simulink model "ex_model_comparison"  (R2026b)
settings: Solver=ode23t  StopTime=2  MaxStep=1e-4  RelTol=1e-5
undefined symbols (not defined in the file or in its folder): L1, L2, L3, Rechtsdrehfeld
libraries: asm_blocks_lib x26, nesl_utility x2
settings Model: Creator=fsbb  LastModifiedBy=fsbb
settings SimscapeCC: SimscapeLogType=all  SimscapeNominalValues="[{\"value\":\"1\",\"unit\":\"A\"},{\"value\":\"1\",\"unit\":\"bar\"},{\"value\":\"1\",\"unit\":\"cm^2\"},{\"value\":\"1\",\"unit\":\"cm^3/s\"},{\"value\":\"1\",\"unit\":\"kJ/kg\"},{\"value\":\"1\",\"unit\":\"kW\"},{\"value\":\"1\",\"unit\":\"l\"},{\"value\":\"1\",\"unit\":\"N\"},{\"value\":\"1\",\"unit\":\"N*m\"},{\"value\":\"1\",\"unit\":\"V\"},{\"value\":\"0.001\",\"unit\":\"Wb\"}]"  SimscapeUseEnergyAccounting=off

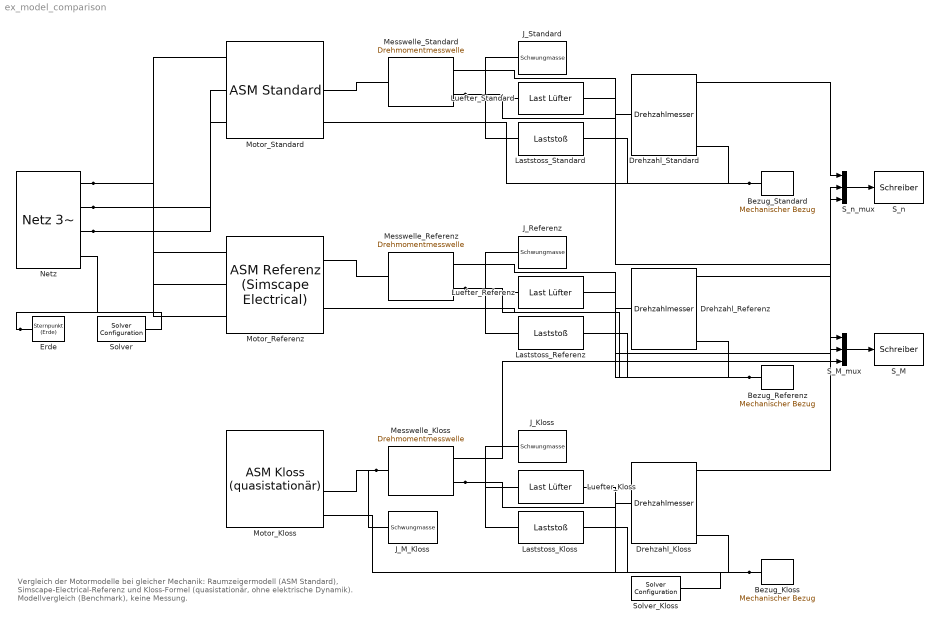
== system ex_model_comparison ==
  note: Vergleich der Motormodelle bei gleicher Mechanik: Raumzeigermodell (ASM Standard), Simscape-Electrical-Referenz und Kloss-Formel (quasistationär, ohne elektrische Dynamik). Modellvergleich (Benchmark), keine Messung.
  Bezug_Kloss : asm_blocks_lib/Mechanik/Mechanischer Bezug  Tag=asmlib:mech_reference
  Bezug_Referenz : asm_blocks_lib/Mechanik/Mechanischer Bezug  Tag=asmlib:mech_reference
  Bezug_Standard : asm_blocks_lib/Mechanik/Mechanischer Bezug  Tag=asmlib:mech_reference
  Drehzahl_Kloss : asm_blocks_lib/Messgeräte/Drehzahlmesser  Tag=asmlib:speed_sensor  ns=1500
  Drehzahl_Referenz : asm_blocks_lib/Messgeräte/Drehzahlmesser  Tag=asmlib:speed_sensor  ns=1500
  Drehzahl_Standard : asm_blocks_lib/Messgeräte/Drehzahlmesser  Tag=asmlib:speed_sensor  ns=1500
  Erde : asm_blocks_lib/Quellen/Sternpunkt (Erde)  Tag=asmlib:neutral_ground
  J_Kloss : asm_blocks_lib/Mechanik/Schwungmasse  Tag=asmlib:inertia  J=0.01  n0=0
  J_M_Kloss : asm_blocks_lib/Mechanik/Schwungmasse  Tag=asmlib:inertia  J=0.012  n0=0
  J_Referenz : asm_blocks_lib/Mechanik/Schwungmasse  Tag=asmlib:inertia  J=0.01  n0=0
  J_Standard : asm_blocks_lib/Mechanik/Schwungmasse  Tag=asmlib:inertia  J=0.01  n0=0
  Laststoss_Kloss : asm_blocks_lib/Mechanik/Laststoß  Tag=asmlib:load_step  t_step=1  dM_L=7.95
  Laststoss_Referenz : asm_blocks_lib/Mechanik/Laststoß  Tag=asmlib:load_step  t_step=1  dM_L=7.95
  Laststoss_Standard : asm_blocks_lib/Mechanik/Laststoß  Tag=asmlib:load_step  t_step=1  dM_L=7.95
  Luefter_Kloss : asm_blocks_lib/Mechanik/Last Lüfter  Tag=asmlib:load_fan  M_B=26.5  n_B=1440
  Luefter_Referenz : asm_blocks_lib/Mechanik/Last Lüfter  Tag=asmlib:load_fan  M_B=26.5  n_B=1440
  Luefter_Standard : asm_blocks_lib/Mechanik/Last Lüfter  Tag=asmlib:load_fan  M_B=26.5  n_B=1440
  Messwelle_Kloss : asm_blocks_lib/Messgeräte/Drehmomentmesswelle  Tag=asmlib:torque_sensor
  Messwelle_Referenz : asm_blocks_lib/Messgeräte/Drehmomentmesswelle  Tag=asmlib:torque_sensor
  Messwelle_Standard : asm_blocks_lib/Messgeräte/Drehmomentmesswelle  Tag=asmlib:torque_sensor
  Motor_Kloss : asm_blocks_lib/Referenz/ASM Kloss (quasistationär)  Tag=asmlib:asm_kloss  MK=71.55  sK=0.2  ns=1500
  Motor_Referenz : asm_blocks_lib/Referenz/ASM Referenz (Simscape Electrical)  Tag=asmlib:asm_reference  param_set=Standard  U_N=400  f_N=50  p=2  R1=0.5  L1s=0.009902  Lh=0.25  R2b=1.225  L2sb=0.009902  J_M=0.012
  Motor_Standard : asm_blocks_lib/Maschine/ASM Standard  Tag=asmlib:asm_standard  param_set=Standard  connection=Stern  U_N=400  f_N=50  p=2  R1=0.5  L1s=0.009902  Lh=0.25  R2b=1.225  L2sb=0.009902  J_M=0.012  k_R=0  n0=0  l=0.15  r=0.06  N2=28  Bhat_N=0.8
  Netz : asm_blocks_lib/Quellen/Netz 3~  Tag=asmlib:grid3  U_L=400  f1=50  phase_seq=L1-L2-L3 (Rechtsdrehfeld)  phi0=0  t_on=0  R_N=0  L_N=0
  S_M : asm_blocks_lib/Messgeräte/Schreiber  Tag=asmlib:recorder  title_text=Wellenmoment: Standard / Referenz / Kloss
  S_M_mux : Mux  Inputs=3
  S_n : asm_blocks_lib/Messgeräte/Schreiber  Tag=asmlib:recorder  title_text=Drehzahl: Standard / Referenz / Kloss
  S_n_mux : Mux  Inputs=3
  Solver : nesl_utility/Solver Configuration  PhysicalDomain=network_engine_domain  SubClassName=solver  LeftPortType=input  RightPortType=generic  Tones=[]  Harmonics=[]  SimulateNoise=off  Profile=off  UseLocalSampling=off  EnableSwitchedLinearOptims=on  FrequencyDomain=off  UseCCode=off  RelTol=0.001  AbsTol=0.001  MinStep=1e-09  ToWorkspace=off  RevertToSquareIcSolve=off  NumHomotopyIterations=100  PhasorMode=off  PhasorModeNumHarmonics=1  ConsistencySolver=NEWTON_XTOL_AFTER_FTOL  CanonicalOrdering=CANONICAL  OptimizeIntermediates=OPTIMIZED  MulticoreSolverChoice=BACKWARD_EULER  IndexReductionMethod=DerivativeReplacement  DoDC=off  ResidualTolerance=1e-09  ConsistencyTolSource=GLOBAL  ConsistencyAbsTol=0.001  ConsistencyRelTol=0.001  ConsistencyTolFactor=0.001  UseLocalSolver=off  LocalSolverChoice=NE_BACKWARD_EULER_ADVANCER  ResolveIndetEquations=on  FunctionEvalNumThread=1  LocalSolverSampleTime=0.001  DoFixedCost=off  MaxNonlinIter=3  MaxModeIter=2  ComputeImpulses=off  ImpulseIterations=2  LinearAlgebra=auto  LinearAlgebraNumThread=0  EquationFormulation=NE_TIME_EF  DelaysMemoryBudget=1024  AutomaticFiltering=on  FilteringTimeConstant=0.001  PartitionStorageMethod=AS_NEEDED  PartitionMemoryBudget=1024  PartitionMethod=BALANCED  MultibodyUseLocalSolver=off  MultibodyLocalSolverChoice=ODE1  MultibodyLocalSolverSampleTime=0.001
  Solver_Kloss : nesl_utility/Solver Configuration  PhysicalDomain=network_engine_domain  SubClassName=solver  LeftPortType=input  RightPortType=generic  Tones=[]  Harmonics=[]  SimulateNoise=off  Profile=off  UseLocalSampling=off  EnableSwitchedLinearOptims=on  FrequencyDomain=off  UseCCode=off  RelTol=0.001  AbsTol=0.001  MinStep=1e-09  ToWorkspace=off  RevertToSquareIcSolve=off  NumHomotopyIterations=100  PhasorMode=off  PhasorModeNumHarmonics=1  ConsistencySolver=NEWTON_XTOL_AFTER_FTOL  CanonicalOrdering=CANONICAL  OptimizeIntermediates=OPTIMIZED  MulticoreSolverChoice=BACKWARD_EULER  IndexReductionMethod=DerivativeReplacement  DoDC=off  ResidualTolerance=1e-09  ConsistencyTolSource=GLOBAL  ConsistencyAbsTol=0.001  ConsistencyRelTol=0.001  ConsistencyTolFactor=0.001  UseLocalSolver=off  LocalSolverChoice=NE_BACKWARD_EULER_ADVANCER  ResolveIndetEquations=on  FunctionEvalNumThread=1  LocalSolverSampleTime=0.001  DoFixedCost=off  MaxNonlinIter=3  MaxModeIter=2  ComputeImpulses=off  ImpulseIterations=2  LinearAlgebra=auto  LinearAlgebraNumThread=0  EquationFormulation=NE_TIME_EF  DelaysMemoryBudget=1024  AutomaticFiltering=on  FilteringTimeConstant=0.001  PartitionStorageMethod=AS_NEEDED  PartitionMemoryBudget=1024  PartitionMethod=BALANCED  MultibodyUseLocalSolver=off  MultibodyLocalSolverChoice=ODE1  MultibodyLocalSolverSampleTime=0.001
  wires:
  Drehzahl_Standard/1 -> S_n_mux/1
  Drehzahl_Referenz/1 -> S_n_mux/2
  Drehzahl_Kloss/1 -> S_n_mux/3
  S_n_mux/1 -> S_n/1
  Messwelle_Standard/1 -> S_M_mux/1
  Messwelle_Referenz/1 -> S_M_mux/2
  Messwelle_Kloss/1 -> S_M_mux/3
  S_M_mux/1 -> S_M/1
  connections:
  Erde/LConn1 -- Netz/RConn4 -- Solver/RConn1
  Motor_Standard/LConn1 -- Netz/RConn1 -- Motor_Referenz/LConn1
  Motor_Standard/LConn2 -- Netz/RConn2 -- Motor_Referenz/LConn2
  Motor_Standard/LConn3 -- Netz/RConn3 -- Motor_Referenz/LConn3
  Motor_Standard/RConn1 -- Messwelle_Standard/LConn1
  Motor_Standard/RConn2 -- Luefter_Standard/RConn1 -- Laststoss_Standard/RConn1 -- Bezug_Standard/LConn1 -- Drehzahl_Standard/RConn1
  J_Standard/LConn1 -- Messwelle_Standard/RConn1 -- Luefter_Standard/LConn1 -- Laststoss_Standard/LConn1 -- Drehzahl_Standard/LConn1
  Motor_Referenz/RConn1 -- Messwelle_Referenz/LConn1
  Motor_Referenz/RConn2 -- Luefter_Referenz/RConn1 -- Laststoss_Referenz/RConn1 -- Bezug_Referenz/LConn1 -- Drehzahl_Referenz/RConn1
  J_Referenz/LConn1 -- Messwelle_Referenz/RConn1 -- Luefter_Referenz/LConn1 -- Laststoss_Referenz/LConn1 -- Drehzahl_Referenz/LConn1
  Messwelle_Kloss/LConn1 -- J_M_Kloss/LConn1 -- Motor_Kloss/RConn1
  Solver_Kloss/RConn1 -- Motor_Kloss/RConn2 -- Luefter_Kloss/RConn1 -- Laststoss_Kloss/RConn1 -- Bezug_Kloss/LConn1 -- Drehzahl_Kloss/RConn1
  J_Kloss/LConn1 -- Messwelle_Kloss/RConn1 -- Luefter_Kloss/LConn1 -- Laststoss_Kloss/LConn1 -- Drehzahl_Kloss/LConn1
